simulink model "hopper_6dof_NED_v2_simplified"  (R2026a)
settings: Solver=FixedStepAuto  StopTime=30  FixedStep=1e-3  RelTol=1e-5
InitFcn:
  | % Feature toggles (1 = on, 0 = off). If no setup script defined them, default to
  | % full physics so this model always compiles and never silently drops physics.
  | % To turn a feature off for one run, prefer Simulink.SimulationInput.setVariable.
  | if ~exist('enable_slosh', 'var'), enable_slosh = 1; end
  | if ~exist('enable_wind', 'var'),  enable_wind  = 1; end
undefined symbols (not defined in the file): cg_init, dcg_dMfu_table, dcg_dMox_table, dI_dMfu_table, dI_dMox_table, ENGINE, engine_cg, engine_mass, fu_axial_damping_ratios, fu_lateral_damping_ratios, fu_mass_profile, fu_masses, fu_mdot_data, g, IN, K1flat, K2grid, MoI_init, mount_cg, OUT, ox_axial_damping_ratios, ox_lateral_damping_ratios, ox_mass_profile, ox_masses, ox_mdot_data, pressureLevels, r_leg_1, r_leg_2, r_leg_3, r_leg_4, tank_r, TANKS, Target_Trajectory, tgrid, thrust_data, unom, uwndTable, VEH, vwndTable
libraries: fl_lib x31, nesl_utility x25, matrix_library x18, SimscapeFluids_lib x10, simulink_extras x7, slpidlib x7, simulink x5, dspindex x3, sl_discontinuities x2, aerolibanim x1, commrandsrc3 x1, dspsrcs4 x1
(part 6 of 7)

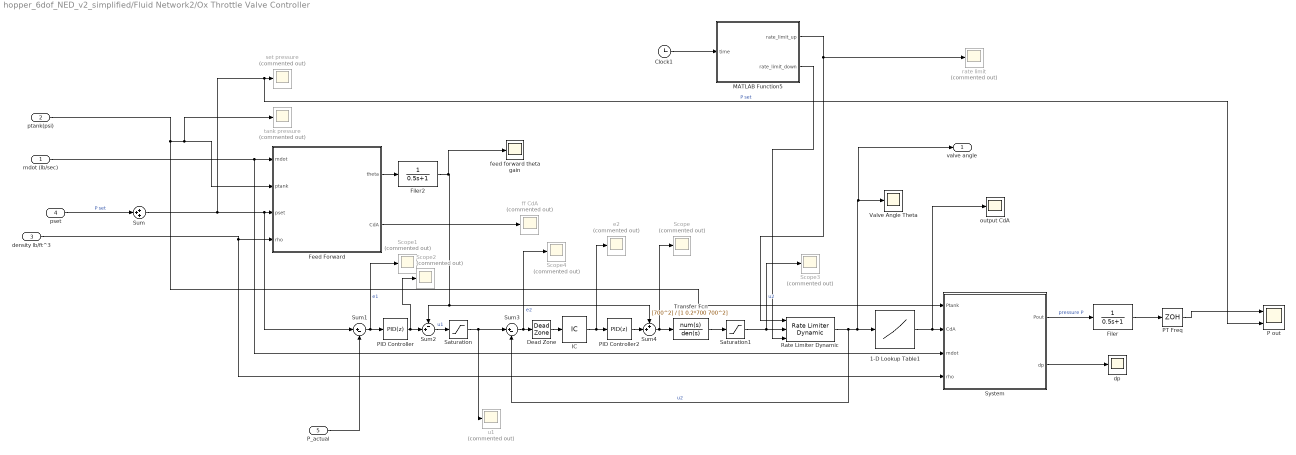
== system hopper_6dof_NED_v2_simplified/Fluid Network2/Ox Throttle Valve Controller ==
  mdot (lb/sec) : Inport
  ptank(psi) : Inport  Port=2
  density lb/ft^3 : Inport  Port=3
  pset : Inport  Port=4
  P_actual : Inport  Port=5
  1-D Lookup Table1 : Lookup_n-D  NumberOfTableDimensions=1  BreakpointsForDimension1=[27, 36, 45, 54, 63, 72, 81, 90]  Table="[0.01,  0.06, 0.21, 0.46, 0.83, 1.35, 2.04, 2.93] ./ 37.97"  ExtrapMethod=Clip  InternalRulePriority=Speed  RndMeth=Simplest
  Clock1 : Clock
  Dead Zone : DeadZone  LowerValue=-30  UpperValue=30
  Feed Forward : MATLAB Function  TreatAsAtomicUnit=on
  Filer : TransferFcn  Denominator=[0.5 1]
  Filer2 : TransferFcn  Denominator=[0.5 1]
  IC : InitialCondition  Value=0
  MATLAB Function5 : MATLAB Function  TreatAsAtomicUnit=on
  P out : Scope  NumInputPorts=2
      settings: ActiveDisplayYMinimum=-153.57845403205533  ActiveDisplayYMaximum=515.02423080214487  DataLoggingVariableName=ScopeData20
  PID Controller : slpidlib/PID Controller  Controller=PID  Form=Parallel  TimeDomain=Discrete-time  UseExternalTs=off  SampleTime=0.01  IntegratorMethod=Forward Euler  FilterMethod=Forward Euler  ControllerParametersSource=internal  P=6  I=0.5  UseKiTs=off  D=0  UseExternalDerivativeSource=off  N=100  UseFilter=on  TunerSelectOption=Transfer Function Based (PID Tuner App)  InitialConditionSource=internal  InitialConditionForIntegrator=0  InitialConditionForFilter=0  DifferentiatorICPrevScaledInput=0  ExternalReset=none  TrackingMode=off  Kt=1  LimitOutput=off  SatLimitsSource=internal  UpperSaturationLimit=inf  LowerSaturationLimit=-inf  LinearizeAsGain=on  AntiWindupMode=none  Kb=1  LimitIntegrator=off  UpperIntegratorSaturationLimit=inf  LowerIntegratorSaturationLimit=-inf  POutMin=[]  POutMax=[]  IOutMin=[]  IOutMax=[]  DOutMin=[]  DOutMax=[]  NOutMin=[]  NOutMax=[]  SumOutMin=[]  SumOutMax=[]  SaturationOutMin=[]  SaturationOutMax=[]  PParamMin=[]  PParamMax=[]  IParamMin=[]  IParamMax=[]  DParamMin=[]  DParamMax=[]  NParamMin=[]  NParamMax=[]  KbParamMin=[]  KbParamMax=[]  KtParamMin=[]  KtParamMax=[]  KbOutMin=[]  KbOutMax=[]  KtOutMin=[]  KtOutMax=[]  IntegratorOutMin=[]  IntegratorOutMax=[]  FilterOutMin=[]  FilterOutMax=[]  SumI1OutMin=[]  SumI1OutMax=[]  SumI2OutMin=[]  SumI2OutMax=[]  SumI3OutMin=[]  SumI3OutMax=[]  SumI4OutMin=[]  SumI4OutMax=[]  SumDOutMin=[]  SumDOutMax=[]  DifferentiatorOutMin=[]  DifferentiatorOutMax=[]  FilterDiffOutCoefMin=[]  FilterDiffOutCoefMax=[]  ReciprocalOutMin=[]  ReciprocalOutMax=[]  SumDenOutMin=[]  SumDenOutMax=[]  SumNumOutMin=[]  SumNumOutMax=[]  DivideOutMin=[]  DivideOutMax=[]  UdiffTsProdOutMin=[]  UdiffTsProdOutMax=[]  NTsProdOutMin=[]  NTsProdOutMax=[]  UintegralTsProdOutMin=[]  UintegralTsProdOutMax=[]  UngainTsProdOutMin=[]  UngainTsProdOutMax=[]  ClampingZeroOutDataTypeStr=Inherit: Inherit via back propagation  ClampingZeroOutMin=[]  ClampingZeroOutMax=[]  FilterDenConstantOutDataTypeStr=Inherit: Inherit via back propagation  FilterDenConstantOutMin=[]  FilterDenConstantOutMax=[]  PCopyOutDataTypeStr=Inherit: Inherit via back propagation  PCopyOutMin=[]  PCopyOutMax=[]  NCopyOutDataTypeStr=Inherit: Inherit via back propagation  NCopyOutMin=[]  NCopyOutMax=[]  IntegratorContinuousStateAttributes=''  IntegratorStateMustResolveToSignalObject=off  IntegratorRTWStateStorageClass=Auto  FilterContinuousStateAttributes=''  FilterStateMustResolveToSignalObject=off  FilterRTWStateStorageClass=Auto  ParallelPVariant=InternalParameters  IdealPVariant=Disabled  IVariant=InternalParameters  DVariant=InternalParameters  IntegratorVariant=Discrete  SatVariant=Disabled  AWVariant=Passthrough  PCopyVariant=Disabled  TRVariant=Disabled  FdbkBlocksVariant=Forward  IdealPFdbkVariant=Disabled  SatFdbkVariant=Disabled  DerivativeFilterVariant=ForwardEulerFilter  NVariant=InternalParameters  NCopyVariant=Disabled  FilterICVariant=InternalICsFilter  IntegratorICVariant=InternalICs  ExternalResetVariant=Disabled  TRSumVariant=Passthrough  SumFdbkVariant=Disabled  SumVariant=Sum_PID  TsampFilterVariant=InternalTs  TsampNgainVariant=Passthrough  TsampIntegralVariant=Disabled_SignalSpec  ExternalSaturationOutDataTypeStr=Inherit: Same as second input  DerivativeSourceVariant=ErrorSignal  PreIntVariant=InternalPreInt
  PID Controller2 : slpidlib/PID Controller  Controller=PID  Form=Parallel  TimeDomain=Discrete-time  UseExternalTs=off  SampleTime=0.001  IntegratorMethod=Forward Euler  FilterMethod=Forward Euler  ControllerParametersSource=internal  P=0.1  I=0.6  UseKiTs=off  D=0  UseExternalDerivativeSource=off  N=100  UseFilter=on  TunerSelectOption=Transfer Function Based (PID Tuner App)  InitialConditionSource=internal  InitialConditionForIntegrator=0  InitialConditionForFilter=0  DifferentiatorICPrevScaledInput=0  ExternalReset=none  TrackingMode=off  Kt=1  LimitOutput=off  SatLimitsSource=internal  UpperSaturationLimit=inf  LowerSaturationLimit=-inf  LinearizeAsGain=on  AntiWindupMode=none  Kb=1  LimitIntegrator=off  UpperIntegratorSaturationLimit=inf  LowerIntegratorSaturationLimit=-inf  POutMin=[]  POutMax=[]  IOutMin=[]  IOutMax=[]  DOutMin=[]  DOutMax=[]  NOutMin=[]  NOutMax=[]  SumOutMin=[]  SumOutMax=[]  SaturationOutMin=[]  SaturationOutMax=[]  PParamMin=[]  PParamMax=[]  IParamMin=[]  IParamMax=[]  DParamMin=[]  DParamMax=[]  NParamMin=[]  NParamMax=[]  KbParamMin=[]  KbParamMax=[]  KtParamMin=[]  KtParamMax=[]  KbOutMin=[]  KbOutMax=[]  KtOutMin=[]  KtOutMax=[]  IntegratorOutMin=[]  IntegratorOutMax=[]  FilterOutMin=[]  FilterOutMax=[]  SumI1OutMin=[]  SumI1OutMax=[]  SumI2OutMin=[]  SumI2OutMax=[]  SumI3OutMin=[]  SumI3OutMax=[]  SumI4OutMin=[]  SumI4OutMax=[]  SumDOutMin=[]  SumDOutMax=[]  DifferentiatorOutMin=[]  DifferentiatorOutMax=[]  FilterDiffOutCoefMin=[]  FilterDiffOutCoefMax=[]  ReciprocalOutMin=[]  ReciprocalOutMax=[]  SumDenOutMin=[]  SumDenOutMax=[]  SumNumOutMin=[]  SumNumOutMax=[]  DivideOutMin=[]  DivideOutMax=[]  UdiffTsProdOutMin=[]  UdiffTsProdOutMax=[]  NTsProdOutMin=[]  NTsProdOutMax=[]  UintegralTsProdOutMin=[]  UintegralTsProdOutMax=[]  UngainTsProdOutMin=[]  UngainTsProdOutMax=[]  ClampingZeroOutDataTypeStr=Inherit: Inherit via back propagation  ClampingZeroOutMin=[]  ClampingZeroOutMax=[]  FilterDenConstantOutDataTypeStr=Inherit: Inherit via back propagation  FilterDenConstantOutMin=[]  FilterDenConstantOutMax=[]  PCopyOutDataTypeStr=Inherit: Inherit via back propagation  PCopyOutMin=[]  PCopyOutMax=[]  NCopyOutDataTypeStr=Inherit: Inherit via back propagation  NCopyOutMin=[]  NCopyOutMax=[]  IntegratorContinuousStateAttributes=''  IntegratorStateMustResolveToSignalObject=off  IntegratorRTWStateStorageClass=Auto  FilterContinuousStateAttributes=''  FilterStateMustResolveToSignalObject=off  FilterRTWStateStorageClass=Auto  ParallelPVariant=InternalParameters  IdealPVariant=Disabled  IVariant=InternalParameters  DVariant=InternalParameters  IntegratorVariant=Discrete  SatVariant=Disabled  AWVariant=Passthrough  PCopyVariant=Disabled  TRVariant=Disabled  FdbkBlocksVariant=Forward  IdealPFdbkVariant=Disabled  SatFdbkVariant=Disabled  DerivativeFilterVariant=ForwardEulerFilter  NVariant=InternalParameters  NCopyVariant=Disabled  FilterICVariant=InternalICsFilter  IntegratorICVariant=InternalICs  ExternalResetVariant=Disabled  TRSumVariant=Passthrough  SumFdbkVariant=Disabled  SumVariant=Sum_PID  TsampFilterVariant=InternalTs  TsampNgainVariant=Passthrough  TsampIntegralVariant=Disabled_SignalSpec  ExternalSaturationOutDataTypeStr=Inherit: Same as second input  DerivativeSourceVariant=ErrorSignal  PreIntVariant=InternalPreInt
  PT Freq : ZeroOrderHold  SampleTime=1/200
  Rate Limiter Dynamic : sl_discontinuities/Rate Limiter Dynamic
  Saturation : Saturate  UpperLimit=90  LowerLimit=0
  Saturation1 : Saturate  UpperLimit=90  LowerLimit=0
  Scope{,1..4} (5 alike) : Scope  Commented=on
      Scope settings: ActiveDisplayYMinimum=-275.11641924282065  ActiveDisplayYMaximum=563.35245614782866  DataLoggingVariableName=ScopeData23
      Scope1 settings: ActiveDisplayYMinimum=-63.640747784829  ActiveDisplayYMaximum=395.9600830872032  DataLoggingVariableName=ScopeData24
      Scope2 settings: ActiveDisplayYMinimum=-1  ActiveDisplayYMaximum=1  DataLoggingVariableName=ScopeData25
      Scope3 settings: ActiveDisplayYMinimum=-1  ActiveDisplayYMaximum=1  DataLoggingVariableName=ScopeData26
      Scope4 settings: ActiveDisplayYMinimum=-1  ActiveDisplayYMaximum=1  DataLoggingVariableName=ScopeData27
  Sum : Sum  Inputs=+++
  Sum1 : Sum  Inputs=|+-
  Sum2 : Sum  Inputs=-+|
  Sum3 : Sum  Inputs=|+-
  Sum4 : Sum  Inputs=++|
  System : MATLAB Function  TreatAsAtomicUnit=on
  Transfer Fcn : TransferFcn  Numerator=[700^2]  Denominator=[1 0.2*700 700^2]
  Valve Angle Theta : Scope
      settings: ActiveDisplayYMinimum=-54.50975234839  ActiveDisplayYMaximum=77.0496336171224
  dp : Scope
      settings: ActiveDisplayYMinimum=-18119.240749435841  ActiveDisplayYMaximum=163753.70976632342  DataLoggingVariableName=ScopeData28
  e2 : Scope  Commented=on
      settings: ActiveDisplayYMinimum=-94.713391249832966  ActiveDisplayYMaximum=253.61308310962266  DataLoggingVariableName=ScopeData29
  feed forward theta gain : Scope
      settings: ActiveDisplayYMinimum=36.144112332478429  ActiveDisplayYMaximum=40.8018145520034  DataLoggingVariableName=ScopeData2
  ff CdA : Scope  Commented=on
      settings: ActiveDisplayYMinimum=0.00619  ActiveDisplayYMaximum=0.00757  DataLoggingVariableName=ScopeData30
  output CdA : Scope
      settings: ActiveDisplayYMinimum=-0.0014226243070618195  ActiveDisplayYMaximum=0.015437276914728357  DataLoggingVariableName=ScopeData3
  rate limit : Scope  Commented=on
      settings: ActiveDisplayYMinimum=-1  ActiveDisplayYMaximum=1  DataLoggingVariableName=ScopeData31
  set pressure : Scope  Commented=on
      settings: ActiveDisplayYMinimum=-1  ActiveDisplayYMaximum=1  DataLoggingVariableName=ScopeData32
  tank pressure : Scope  Commented=on
      settings: ActiveDisplayYMinimum=243.75  ActiveDisplayYMaximum=306.25  DataLoggingVariableName=ScopeData33
  u1 : Scope  Commented=on
      settings: ActiveDisplayYMinimum=-1  ActiveDisplayYMaximum=1  DataLoggingVariableName=ScopeData34
  valve angle : Outport
  wires:
  Sum3/1 -> Dead Zone/1, Scope4/1  "e2"
  density lb/ft^3/1 -> System/4(rho), Feed Forward/4(rho)
  Filer/1 -> PT Freq/1
  Sum/1 -> P out/2, set pressure/1, Sum1/1, Feed Forward/3(pset)  "P set"
  ptank(psi)/1 -> System/1(Ptank), Feed Forward/2(ptank), tank pressure/1
  PID Controller/1 -> Scope2/1, Sum2/2
  PT Freq/1 -> P out/1
  Transfer Fcn/1 -> Saturation1/1
  IC/1 -> PID Controller2/1, e2/1
  Feed Forward/1(theta) -> Filer2/1
  MATLAB Function5/2(rate_limit_down) -> Rate Limiter Dynamic/3
  Dead Zone/1 -> IC/1
  Rate Limiter Dynamic/1 -> valve angle/1, Valve Angle Theta/1, 1-D Lookup Table1/1, Sum3/2  "u2"
  pset/1 -> Sum/2  "P set"
  Sum4/1 -> Scope/1, Transfer Fcn/1
  Saturation1/1 -> Scope3/1, Rate Limiter Dynamic/2  "u2"
  mdot (lb/sec)/1 -> System/3(mdot), Feed Forward/1(mdot)
  MATLAB Function5/1(rate_limit_up) -> Rate Limiter Dynamic/1, rate limit/1
  Clock1/1 -> MATLAB Function5/1(time)
  1-D Lookup Table1/1 -> System/2(CdA), output CdA/1
  PID Controller2/1 -> Sum4/2
  Sum1/1 -> Scope1/1, PID Controller/1  "e1"
  Sum2/1 -> Saturation/1  "u1"
  Feed Forward/2(CdA) -> ff CdA/1
  System/2(dp) -> dp/1
  Saturation/1 -> u1/1, Sum3/1
  System/1(Pout) -> Filer/1  "pressure P"
  Filer2/1 -> Sum4/1, Sum2/1, feed forward theta gain/1
  P_actual/1 -> Sum1/2

== system hopper_6dof_NED_v2_simplified/Fluid Network2/Physical Combustion Chamber ==
  pc : Inport
  Local Restriction (TL) : fl_lib/Thermal Liquid/Elements/Local Restriction (TL)  Commented=through  restriction_type=foundation.enum.restriction_type.fixed  restriction_area=0.001 m^2  min_area=1e-10 m^2  max_area=0.005 m^2  area=0.01 m^2  Cd=0.64  Re_c=150  pressure_recovery=true
  Local Restriction (TL)1 : fl_lib/Thermal Liquid/Elements/Local Restriction (TL)  Commented=through  restriction_type=foundation.enum.restriction_type.fixed  restriction_area=0.001 m^2  min_area=1e-10 m^2  max_area=0.005 m^2  area=0.01 m^2  Cd=0.64  Re_c=150  pressure_recovery=true
  Pressure Source (TL) : fl_lib/Thermal Liquid/Sources/Pressure Source (TL)  source_type=foundation.enum.constant_controlled.controlled  pressure_differential=0 MPa  power_spec=foundation.enum.power_spec.isentropic  area=0.01 m^2
  Pressure Source (TL)1 : fl_lib/Thermal Liquid/Sources/Pressure Source (TL)  source_type=foundation.enum.constant_controlled.controlled  pressure_differential=0 MPa  power_spec=foundation.enum.power_spec.isentropic  area=0.01 m^2
  Reservoir (TL) : fl_lib/Thermal Liquid/Elements/Reservoir (TL)  pressure_input=false  pressure_spec=foundation.enum.pressure_spec.atmospheric  reservoir_pressure=0.101325 MPa  temperature_input=false  reservoir_temperature=293.15 K  area=0.01 m^2  input_error_spec=foundation.enum.input_range_error.warn
  Reservoir (TL)1 : fl_lib/Thermal Liquid/Elements/Reservoir (TL)  pressure_input=false  pressure_spec=foundation.enum.pressure_spec.atmospheric  reservoir_pressure=0.101325 MPa  temperature_input=false  reservoir_temperature=100 K  area=0.01 m^2  input_error_spec=foundation.enum.input_range_error.warn
  Simulink-PS Converter1 : nesl_utility/Simulink-PS Converter  PhysicalDomain=network_engine_domain  SubClassName=ps_input  LeftPortType=input  RightPortType=output  PseudoPeriodic=off  Frequencies=[]  NoiseDistribution=none  NoiseParameters=[]  Unit=1  AffineConversion=off  FilteringAndDerivatives=filter  SimscapeFilterOrder=1  InputFilterTimeConstant=0.001  UdotUserProvided=0
  Simulink-PS Converter4 : nesl_utility/Simulink-PS Converter  PhysicalDomain=network_engine_domain  SubClassName=ps_input  LeftPortType=input  RightPortType=output  PseudoPeriodic=off  Frequencies=[]  NoiseDistribution=none  NoiseParameters=[]  Unit=1  AffineConversion=off  FilteringAndDerivatives=filter  SimscapeFilterOrder=1  InputFilterTimeConstant=0.001  UdotUserProvided=0
  fuel line : PMIOPort  Side=Right
  ox line : PMIOPort  Port=2  Side=Right
  wires:
  pc/1 -> Simulink-PS Converter1/1, Simulink-PS Converter4/1
  connections:
  Simulink-PS Converter4/RConn1 -- Pressure Source (TL)/LConn2
  Simulink-PS Converter1/RConn1 -- Pressure Source (TL)1/LConn2
  Local Restriction (TL)/LConn1 -- Pressure Source (TL)/LConn1
  Reservoir (TL)/LConn1 -- Local Restriction (TL)/RConn1
  fuel line/RConn1 -- Pressure Source (TL)/RConn1
  Local Restriction (TL)1/LConn1 -- Pressure Source (TL)1/LConn1
  Reservoir (TL)1/LConn1 -- Local Restriction (TL)1/RConn1
  Pressure Source (TL)1/RConn1 -- ox line/RConn1

== system hopper_6dof_NED_v2_simplified/Fluid Network2/fuel mdot feedback//corrections ==
  actual mdot : Inport
  commanded mdot : Inport  Port=2
  MR correction : Inport  Port=3
  PID Controller1 : slpidlib/PID Controller  Controller=PID  Form=Parallel  TimeDomain=Continuous-time  UseExternalTs=off  SampleTime=-1  IntegratorMethod=Forward Euler  FilterMethod=Forward Euler  ControllerParametersSource=internal  P=1  I=1  UseKiTs=off  D=0  UseExternalDerivativeSource=off  N=20  UseFilter=on  TunerSelectOption=Transfer Function Based (PID Tuner App)  InitialConditionSource=internal  InitialConditionForIntegrator=0  InitialConditionForFilter=0  DifferentiatorICPrevScaledInput=0  ExternalReset=none  TrackingMode=off  Kt=1  LimitOutput=off  SatLimitsSource=internal  UpperSaturationLimit=inf  LowerSaturationLimit=-inf  LinearizeAsGain=on  AntiWindupMode=none  Kb=1  LimitIntegrator=off  UpperIntegratorSaturationLimit=inf  LowerIntegratorSaturationLimit=-inf  POutMin=[]  POutMax=[]  IOutMin=[]  IOutMax=[]  DOutMin=[]  DOutMax=[]  NOutMin=[]  NOutMax=[]  SumOutMin=[]  SumOutMax=[]  SaturationOutMin=[]  SaturationOutMax=[]  PParamMin=[]  PParamMax=[]  IParamMin=[]  IParamMax=[]  DParamMin=[]  DParamMax=[]  NParamMin=[]  NParamMax=[]  KbParamMin=[]  KbParamMax=[]  KtParamMin=[]  KtParamMax=[]  KbOutMin=[]  KbOutMax=[]  KtOutMin=[]  KtOutMax=[]  IntegratorOutMin=[]  IntegratorOutMax=[]  FilterOutMin=[]  FilterOutMax=[]  SumI1OutMin=[]  SumI1OutMax=[]  SumI2OutMin=[]  SumI2OutMax=[]  SumI3OutMin=[]  SumI3OutMax=[]  SumI4OutMin=[]  SumI4OutMax=[]  SumDOutMin=[]  SumDOutMax=[]  DifferentiatorOutMin=[]  DifferentiatorOutMax=[]  FilterDiffOutCoefMin=[]  FilterDiffOutCoefMax=[]  ReciprocalOutMin=[]  ReciprocalOutMax=[]  SumDenOutMin=[]  SumDenOutMax=[]  SumNumOutMin=[]  SumNumOutMax=[]  DivideOutMin=[]  DivideOutMax=[]  UdiffTsProdOutMin=[]  UdiffTsProdOutMax=[]  NTsProdOutMin=[]  NTsProdOutMax=[]  UintegralTsProdOutMin=[]  UintegralTsProdOutMax=[]  UngainTsProdOutMin=[]  UngainTsProdOutMax=[]  ClampingZeroOutDataTypeStr=Inherit: Inherit via back propagation  ClampingZeroOutMin=[]  ClampingZeroOutMax=[]  FilterDenConstantOutDataTypeStr=Inherit: Inherit via back propagation  FilterDenConstantOutMin=[]  FilterDenConstantOutMax=[]  PCopyOutDataTypeStr=Inherit: Inherit via back propagation  PCopyOutMin=[]  PCopyOutMax=[]  NCopyOutDataTypeStr=Inherit: Inherit via back propagation  NCopyOutMin=[]  NCopyOutMax=[]  IntegratorContinuousStateAttributes=''  IntegratorStateMustResolveToSignalObject=off  IntegratorRTWStateStorageClass=Auto  FilterContinuousStateAttributes=''  FilterStateMustResolveToSignalObject=off  FilterRTWStateStorageClass=Auto  ParallelPVariant=InternalParameters  IdealPVariant=Disabled  IVariant=InternalParameters  DVariant=InternalParameters  IntegratorVariant=Continuous  SatVariant=Disabled  AWVariant=Passthrough  PCopyVariant=Disabled  TRVariant=Disabled  FdbkBlocksVariant=Forward  IdealPFdbkVariant=Disabled  SatFdbkVariant=Disabled  DerivativeFilterVariant=ContFilter  NVariant=InternalParameters  NCopyVariant=Disabled  FilterICVariant=InternalICsFilter  IntegratorICVariant=InternalICs  ExternalResetVariant=Disabled  TRSumVariant=Passthrough  SumFdbkVariant=Disabled  SumVariant=Sum_PID  TsampFilterVariant=InternalTs  TsampNgainVariant=Passthrough  TsampIntegralVariant=Disabled_SignalSpec  ExternalSaturationOutDataTypeStr=Inherit: Same as second input  DerivativeSourceVariant=ErrorSignal  PreIntVariant=InternalPreInt
  Sum2 : Sum  Inputs=|+-
  Sum3 : Sum  Inputs=|+-
  Sum4 : Sum  Inputs=|++
  kg/s to lb/s1 : Gain  Gain=2.20462
  fuel mdot : Outport
  wires:
  MR correction/1 -> Sum2/2
  Sum2/1 -> Sum4/2, Sum3/1
  PID Controller1/1 -> Sum4/1
  Sum3/1 -> PID Controller1/1
  Sum4/1 -> kg/s to lb/s1/1
  commanded mdot/1 -> Sum2/1
  actual mdot/1 -> Sum3/2
  kg/s to lb/s1/1 -> fuel mdot/1

== system hopper_6dof_NED_v2_simplified/Fluid Network2/ox mdot feedback//corrections ==
  commanded mdot : Inport
  actual mdot : Inport  Port=2
  PID Controller2 : slpidlib/PID Controller  Controller=PID  Form=Parallel  TimeDomain=Continuous-time  UseExternalTs=off  SampleTime=-1  IntegratorMethod=Forward Euler  FilterMethod=Forward Euler  ControllerParametersSource=internal  P=1  I=1  UseKiTs=off  D=0  UseExternalDerivativeSource=off  N=20  UseFilter=on  TunerSelectOption=Transfer Function Based (PID Tuner App)  InitialConditionSource=internal  InitialConditionForIntegrator=0  InitialConditionForFilter=0  DifferentiatorICPrevScaledInput=0  ExternalReset=none  TrackingMode=off  Kt=1  LimitOutput=off  SatLimitsSource=internal  UpperSaturationLimit=inf  LowerSaturationLimit=-inf  LinearizeAsGain=on  AntiWindupMode=none  Kb=1  LimitIntegrator=off  UpperIntegratorSaturationLimit=inf  LowerIntegratorSaturationLimit=-inf  POutMin=[]  POutMax=[]  IOutMin=[]  IOutMax=[]  DOutMin=[]  DOutMax=[]  NOutMin=[]  NOutMax=[]  SumOutMin=[]  SumOutMax=[]  SaturationOutMin=[]  SaturationOutMax=[]  PParamMin=[]  PParamMax=[]  IParamMin=[]  IParamMax=[]  DParamMin=[]  DParamMax=[]  NParamMin=[]  NParamMax=[]  KbParamMin=[]  KbParamMax=[]  KtParamMin=[]  KtParamMax=[]  KbOutMin=[]  KbOutMax=[]  KtOutMin=[]  KtOutMax=[]  IntegratorOutMin=[]  IntegratorOutMax=[]  FilterOutMin=[]  FilterOutMax=[]  SumI1OutMin=[]  SumI1OutMax=[]  SumI2OutMin=[]  SumI2OutMax=[]  SumI3OutMin=[]  SumI3OutMax=[]  SumI4OutMin=[]  SumI4OutMax=[]  SumDOutMin=[]  SumDOutMax=[]  DifferentiatorOutMin=[]  DifferentiatorOutMax=[]  FilterDiffOutCoefMin=[]  FilterDiffOutCoefMax=[]  ReciprocalOutMin=[]  ReciprocalOutMax=[]  SumDenOutMin=[]  SumDenOutMax=[]  SumNumOutMin=[]  SumNumOutMax=[]  DivideOutMin=[]  DivideOutMax=[]  UdiffTsProdOutMin=[]  UdiffTsProdOutMax=[]  NTsProdOutMin=[]  NTsProdOutMax=[]  UintegralTsProdOutMin=[]  UintegralTsProdOutMax=[]  UngainTsProdOutMin=[]  UngainTsProdOutMax=[]  ClampingZeroOutDataTypeStr=Inherit: Inherit via back propagation  ClampingZeroOutMin=[]  ClampingZeroOutMax=[]  FilterDenConstantOutDataTypeStr=Inherit: Inherit via back propagation  FilterDenConstantOutMin=[]  FilterDenConstantOutMax=[]  PCopyOutDataTypeStr=Inherit: Inherit via back propagation  PCopyOutMin=[]  PCopyOutMax=[]  NCopyOutDataTypeStr=Inherit: Inherit via back propagation  NCopyOutMin=[]  NCopyOutMax=[]  IntegratorContinuousStateAttributes=''  IntegratorStateMustResolveToSignalObject=off  IntegratorRTWStateStorageClass=Auto  FilterContinuousStateAttributes=''  FilterStateMustResolveToSignalObject=off  FilterRTWStateStorageClass=Auto  ParallelPVariant=InternalParameters  IdealPVariant=Disabled  IVariant=InternalParameters  DVariant=InternalParameters  IntegratorVariant=Continuous  SatVariant=Disabled  AWVariant=Passthrough  PCopyVariant=Disabled  TRVariant=Disabled  FdbkBlocksVariant=Forward  IdealPFdbkVariant=Disabled  SatFdbkVariant=Disabled  DerivativeFilterVariant=ContFilter  NVariant=InternalParameters  NCopyVariant=Disabled  FilterICVariant=InternalICsFilter  IntegratorICVariant=InternalICs  ExternalResetVariant=Disabled  TRSumVariant=Passthrough  SumFdbkVariant=Disabled  SumVariant=Sum_PID  TsampFilterVariant=InternalTs  TsampNgainVariant=Passthrough  TsampIntegralVariant=Disabled_SignalSpec  ExternalSaturationOutDataTypeStr=Inherit: Same as second input  DerivativeSourceVariant=ErrorSignal  PreIntVariant=InternalPreInt
  Sum1 : Sum  Inputs=|+-
  Sum5 : Sum  Inputs=|++
  kg/s to lb/s : Gain  Gain=2.20462
  ox mdot : Outport
  wires:
  Sum1/1 -> PID Controller2/1
  commanded mdot/1 -> Sum5/2, Sum1/1
  PID Controller2/1 -> Sum5/1
  Sum5/1 -> kg/s to lb/s/1
  kg/s to lb/s/1 -> ox mdot/1
  actual mdot/1 -> Sum1/2

== system hopper_6dof_NED_v2_simplified/Ground /Leg 1 Force ==
  Leg Position : Inport
  Leg Velocity : Inport  Port=2
  Demux : Demux  Outputs=3
  Demux1 : Demux  Outputs=3
  If : If  NumInputs=2  IfExpression=u1 > -0.001
  If Action Subsystem : Subsystem  TreatAsAtomicUnit=on
  If Action Subsystem1 : Subsystem  TreatAsAtomicUnit=on
  Merge : Merge
  Leg 1 Force : Outport
  wires:
  Leg Position/1 -> If Action Subsystem/1(Leg Position), Demux/1
  If/2 -> If Action Subsystem1/Action
  If Action Subsystem/1(Leg Force) -> Merge/1
  If Action Subsystem1/1(Out1) -> Merge/2
  Merge/1 -> Leg 1 Force/1
  Leg Velocity/1 -> Demux1/1, If Action Subsystem/2(Leg Velocity)
  If/1 -> If Action Subsystem/Action
  Demux/3 -> If/1
  Demux1/3 -> If/2

== system hopper_6dof_NED_v2_simplified/Ground /Leg 1 Force1 ==
  Leg Position : Inport
  Leg Velocity : Inport  Port=2
  Demux : Demux  Outputs=3
  Demux1 : Demux  Outputs=3
  If : If  NumInputs=2  IfExpression=u1 > -0.001
  If Action Subsystem : Subsystem  TreatAsAtomicUnit=on
  If Action Subsystem1 : Subsystem  TreatAsAtomicUnit=on
  Merge : Merge
  Leg 1 Force : Outport
  wires:
  Leg Position/1 -> If Action Subsystem/1(Leg Position), Demux/1
  If/2 -> If Action Subsystem1/Action
  If Action Subsystem/1(Leg Force) -> Merge/1
  If Action Subsystem1/1(Out1) -> Merge/2
  Merge/1 -> Leg 1 Force/1
  Leg Velocity/1 -> Demux1/1, If Action Subsystem/2(Leg Velocity)
  If/1 -> If Action Subsystem/Action
  Demux/3 -> If/1
  Demux1/3 -> If/2

== system hopper_6dof_NED_v2_simplified/Ground /Leg 1 Force2 ==
  Leg Position : Inport
  Leg Velocity : Inport  Port=2
  Demux : Demux  Outputs=3
  Demux1 : Demux  Outputs=3
  If : If  NumInputs=2  IfExpression=u1 > -0.001
  If Action Subsystem : Subsystem  TreatAsAtomicUnit=on
  If Action Subsystem1 : Subsystem  TreatAsAtomicUnit=on
  Merge : Merge
  Leg 1 Force : Outport
  wires:
  Leg Position/1 -> If Action Subsystem/1(Leg Position), Demux/1
  If/2 -> If Action Subsystem1/Action
  If Action Subsystem/1(Leg Force) -> Merge/1
  If Action Subsystem1/1(Out1) -> Merge/2
  Merge/1 -> Leg 1 Force/1
  Leg Velocity/1 -> Demux1/1, If Action Subsystem/2(Leg Velocity)
  If/1 -> If Action Subsystem/Action
  Demux/3 -> If/1
  Demux1/3 -> If/2

== system hopper_6dof_NED_v2_simplified/Ground /Leg 1 Force3 ==
  Leg Position : Inport
  Leg Velocity : Inport  Port=2
  Demux : Demux  Outputs=3
  Demux1 : Demux  Outputs=3
  If : If  NumInputs=2  IfExpression=u1 > -0.001
  If Action Subsystem : Subsystem  TreatAsAtomicUnit=on
  If Action Subsystem1 : Subsystem  TreatAsAtomicUnit=on
  Merge : Merge
  Leg 1 Force : Outport
  wires:
  Leg Position/1 -> If Action Subsystem/1(Leg Position), Demux/1
  If/2 -> If Action Subsystem1/Action
  If Action Subsystem/1(Leg Force) -> Merge/1
  If Action Subsystem1/1(Out1) -> Merge/2
  Merge/1 -> Leg 1 Force/1
  Leg Velocity/1 -> Demux1/1, If Action Subsystem/2(Leg Velocity)
  If/1 -> If Action Subsystem/Action
  Demux/3 -> If/1
  Demux1/3 -> If/2

== system hopper_6dof_NED_v2_simplified/Gusts/Disabled ==
  Zero1 : Constant  Value=0
  Out1 : Outport
  wires:
  Zero1/1 -> Out1/1

== system hopper_6dof_NED_v2_simplified/Gusts/Enabled ==
  Bernoulli Binary Generator : commrandsrc3/Bernoulli Binary Generator  ProbabilityOfZero=0.95  SeedSource=Parameter  Seed=0  SampleTime=0.1  SamplesPerFrame=1  OutputDataType=double  SimulateUsing=Interpreted execution
  Product1 : Product
  Random Source : dspsrcs4/Random Source  SrcType=Gaussian  MinVal=0  MaxVal=1  MeanVal=0  VarVal=20  RepMode=Specify seed  rawSeed=1  IsInherit=off  SampTime=1  SampFrame=1  OutComplex=Real  DataType=double  SimulateUsing=Interpreted execution
  Out1 : Outport
  wires:
  Product1/1 -> Out1/1
  Bernoulli Binary Generator/1 -> Product1/1
  Random Source/1 -> Product1/2

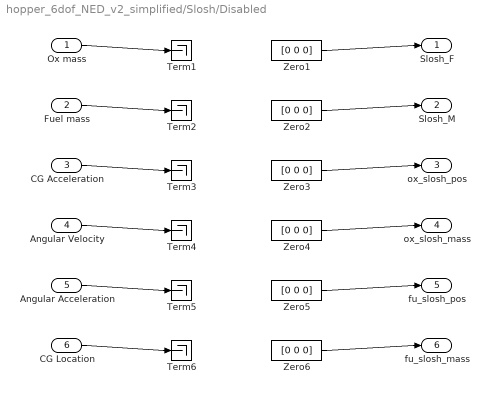
== system hopper_6dof_NED_v2_simplified/Slosh/Disabled ==
  Ox mass : Inport
  Fuel mass : Inport  Port=2
  CG Acceleration : Inport  Port=3
  Angular Velocity : Inport  Port=4
  Angular Acceleration : Inport  Port=5
  CG Location : Inport  Port=6
  Term{1..6} (6 alike) : Terminator
  Zero{1..6} (6 alike) : Constant  Value=[0 0 0]
  Slosh_F : Outport
  Slosh_M : Outport  Port=2
  ox_slosh_pos : Outport  Port=3
  ox_slosh_mass : Outport  Port=4
  fu_slosh_pos : Outport  Port=5
  fu_slosh_mass : Outport  Port=6
  wires:
  Ox mass/1 -> Term1/1
  Fuel mass/1 -> Term2/1
  CG Acceleration/1 -> Term3/1
  Angular Velocity/1 -> Term4/1
  Angular Acceleration/1 -> Term5/1
  CG Location/1 -> Term6/1
  Zero1/1 -> Slosh_F/1
  Zero2/1 -> Slosh_M/1
  Zero3/1 -> ox_slosh_pos/1
  Zero4/1 -> ox_slosh_mass/1
  Zero5/1 -> fu_slosh_pos/1
  Zero6/1 -> fu_slosh_mass/1

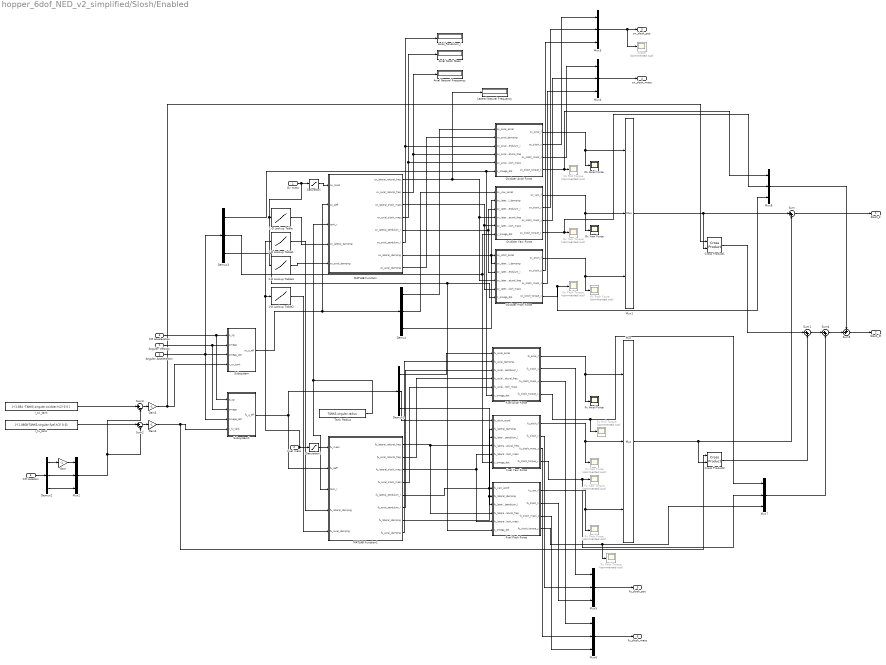
== system hopper_6dof_NED_v2_simplified/Slosh/Enabled ==
  Ox mass : Inport
  Fuel mass : Inport  Port=2
  CG Acceleration : Inport  Port=3
  Angular Velocity : Inport  Port=4
  Angular Acceleration : Inport  Port=5
  CG Location : Inport  Port=6
  1-D Lookup Table : Lookup_n-D  NumberOfTableDimensions=1  BreakpointsForDimension1=ox_mass_profile  Table=ox_lateral_damping_ratios  InternalRulePriority=Speed  RndMeth=Simplest
  1-D Lookup Table1 : Lookup_n-D  NumberOfTableDimensions=1  BreakpointsForDimension1=fu_mass_profile  Table=fu_lateral_damping_ratios  InternalRulePriority=Speed  RndMeth=Simplest
  1-D Lookup Table2 : Lookup_n-D  NumberOfTableDimensions=1  BreakpointsForDimension1=fu_mass_profile  Table=fu_axial_damping_ratios  InternalRulePriority=Speed  RndMeth=Simplest
  1-D Lookup Table4 : Lookup_n-D  NumberOfTableDimensions=1  BreakpointsForDimension1=ox_mass_profile  Table=ox_axial_damping_ratios  InternalRulePriority=Speed  RndMeth=Simplest
  Axial Natural Frequency : Display
  Axial Slosh Mass : Display
  Axial_Pendulum_l : Display
  Cross Product1 : matrix_library/Cross Product
  Cross Product2 : matrix_library/Cross Product
  Demux{,1..3} (4 alike) : Demux  Outputs=3
  Fu Axial Force : Scope
      settings: ActiveDisplayYMinimum=-4.5487995330933861  ActiveDisplayYMaximum=10.430303988696288  DataLoggingVariableName=ScopeData38
  Fu Pitch Force : Scope  Commented=on
      settings: ActiveDisplayYMinimum=-2.9742058993087932  ActiveDisplayYMaximum=15.331760127930639  DataLoggingVariableName=ScopeData40
  Fu Pitch Torque : Scope  Commented=on
      settings: ActiveDisplayYMinimum=-0.19116574787256713  ActiveDisplayYMaximum=0.19970427620804132  DataLoggingVariableName=ScopeData87
  Fu Roll Torque : Scope  Commented=on
      settings: ActiveDisplayYMinimum=-9.5580450498277436  ActiveDisplayYMaximum=8.6061310713641461  DataLoggingVariableName=ScopeData86
  Fu Yaw Force : Scope  Commented=on
      settings: ActiveDisplayYMinimum=-1.96682346554972  ActiveDisplayYMaximum=2.7427386100438831  DataLoggingVariableName=ScopeData39
  Fu Yaw Torque : Scope  Commented=on
      settings: ActiveDisplayYMinimum=-3.6886267521568623  ActiveDisplayYMaximum=3.9647425854021145  DataLoggingVariableName=ScopeData82
  Fuel Axial Force : Subsystem
  Fuel Pitch Force : Subsystem
  Fuel Yaw Force : Subsystem
  Gain : Gain  Gain=-1
  Gain3 : Gain  Gain=-1
  Gain4 : Gain  Gain=-1
  Lateral Natural Frequency : Display
  MATLAB Function : MATLAB Function  TreatAsAtomicUnit=on
  MATLAB Function1 : MATLAB Function  TreatAsAtomicUnit=on
  Mux{,1..8} (9 alike) : Mux  Inputs=3
  Ox Axial Force : Scope
      settings: ActiveDisplayYMinimum=14.43010515330246  ActiveDisplayYMaximum=16.756383333748122  DataLoggingVariableName=ScopeData34
  Ox Pitch Force : Scope  Commented=on
      settings: ActiveDisplayYMinimum=-4.4950785008236629  ActiveDisplayYMaximum=22.001881619828325  DataLoggingVariableName=ScopeData36
  Ox Pitch Torque : Scope  Commented=on
      settings: ActiveDisplayYMinimum=-0.69593653498138675  ActiveDisplayYMaximum=0.79680864639954685  DataLoggingVariableName=ScopeData85
  Ox Roll Torque : Scope  Commented=on
      settings: ActiveDisplayYMinimum=-0.15656949128956149  ActiveDisplayYMaximum=0.79158034254760723  DataLoggingVariableName=ScopeData80
  Ox Yaw Force : Scope
      settings: ActiveDisplayYMinimum=-5.8284827308381395  ActiveDisplayYMaximum=24.723450598791928  DataLoggingVariableName=ScopeData37
  Ox Yaw Torque : Scope  Commented=on
      settings: ActiveDisplayYMinimum=-0.3482323750211066  ActiveDisplayYMaximum=0.31743853430357161  DataLoggingVariableName=ScopeData81
  Oxidizer Axial Force : Subsystem
  Oxidizer Pitch Force : Subsystem
  Oxidizer Yaw Force : Subsystem
  Saturation : Saturate  UpperLimit=inf  LowerLimit=0.01
  Saturation1 : Saturate  UpperLimit=inf  LowerLimit=0.01
  Scope : Scope  Commented=on
      settings: ActiveDisplayYMinimum=-0.0849364779794028  ActiveDisplayYMaximum=0.368207880424993  DataLoggingVariableName=ScopeData35
  Subsystem : Subsystem
  Subsystem1 : Subsystem
  Sum : Sum  Inputs=|++
  Sum1 : Sum  Inputs=|++
  Sum2 : Sum  Inputs=|+-
  Sum3 : Sum  Inputs=|+-
  Sum4 : Sum  Inputs=|++
  Sum5 : Sum  Inputs=++|
  Tank Radius : Constant  Value=TANKS.singular.radius  SampleTime=-1
  r_fu_tank : Constant  Value=[-(1.0668-TANKS.singular.fuel.h/2) 0 0]
  r_ox_tank : Constant  Value=[-(1.854 -TANKS.singular.oxidizer.h/2) 0 0 ]
  Slosh_F : Outport
  Slosh_M : Outport  Port=2
  ox_slosh_pos : Outport  Port=3
  ox_slosh_mass : Outport  Port=4
  fu_slosh_pos : Outport  Port=5
  fu_slosh_mass : Outport  Port=6
  wires:
  1-D Lookup Table2/1 -> MATLAB Function1/5("fu_axial_damping ")
  1-D Lookup Table4/1 -> MATLAB Function/5("ox_axial_damping ")
  1-D Lookup Table1/1 -> MATLAB Function1/4("fu_lateral_damping ")
  1-D Lookup Table/1 -> MATLAB Function/4("ox_lateral_damping ")
  Saturation1/1 -> MATLAB Function1/1(fu_mass)
  Saturation/1 -> MATLAB Function/1(ox_mass)
  Mux7/1 -> Sum4/2
  Mux8/1 -> Sum5/1
  Oxidizer Yaw Force/4(ox_slosh_torque_y) -> Ox Yaw Torque/1, Mux8/2
  Sum4/1 -> Sum5/2
  Sum5/1 -> Slosh_M/1
  Sum1/1 -> Sum4/1
  Oxidizer Pitch Force/4(ox_slosh_torque_z) -> Mux8/3, Ox Pitch Torque/1
  Oxidizer Axial Force/4(ox_slosh_torque_x) -> Ox Roll Torque/1, Mux8/1
  Fuel Pitch Force/4(fu_slosh_torque_z) -> Fu Pitch Torque/1, Mux7/3
  Fuel Yaw Force/4(fu_slosh_torque_y) -> Fu Yaw Torque/1, Mux7/2
  Fuel Axial Force/4(fu_slosh_torque_x) -> Fu Roll Torque/1, Mux7/1
  Demux3/3 -> Oxidizer Pitch Force/6(z_omega_dot), Fuel Pitch Force/6(z_omega_dot)
  Demux3/2 -> Oxidizer Yaw Force/6(y_omega_dot), Fuel Yaw Force/6(y_omega_dot)
  Demux3/1 -> Fuel Axial Force/6(x_omega_dot), Oxidizer Axial Force/6(x_omega_dot)
  Fuel Axial Force/2(fu_slosh_x) -> Mux5/1
  Oxidizer Axial Force/2(ox_slosh_x) -> Mux3/1
  Fuel Pitch Force/3(fu_slosh_mass_z) -> Mux6/3
  Fuel Yaw Force/3(fu_slosh_mass_y) -> Mux6/2
  Fuel Axial Force/3(fu_slosh_mass_x) -> Mux6/1
  Fuel Pitch Force/2(fu_slosh_z) -> Mux5/3
  Fuel Yaw Force/2(fu_slosh_y) -> Mux5/2
  Mux6/1 -> fu_slosh_mass/1
  Mux5/1 -> fu_slosh_pos/1
  Mux4/1 -> ox_slosh_mass/1
  Oxidizer Pitch Force/3(ox_slosh_mass_z) -> Mux4/3
  Oxidizer Pitch Force/2(ox_slosh_z) -> Mux3/3
  Oxidizer Yaw Force/3(ox_slosh_mass_y) -> Mux4/2
  Oxidizer Axial Force/3(ox_slosh_mass_x) -> Mux4/1
  Mux3/1 -> ox_slosh_pos/1, Scope/1
  Oxidizer Yaw Force/2(ox_slosh_y) -> Mux3/2
  Gain/1 -> Mux2/1
  Demux2/1 -> Gain/1
  Demux2/2 -> Mux2/2
  CG Location/1 -> Demux2/1
  Demux2/3 -> Mux2/3
  Gain4/1 -> Subsystem1/4(r_fu_tank), Cross Product2/1
  Gain3/1 -> Subsystem/4(r_ox_tank), Cross Product1/1
  Oxidizer Pitch Force/1(ox_pitch_f) -> Ox Pitch Force/1, Mux1/3
  Fuel Pitch Force/1(fu_yaw_f) -> Fu Pitch Force/1, Mux/3
  Sum2/1 -> Gain4/1
  Sum3/1 -> Gain3/1
  Mux2/1 -> Sum3/2, Sum2/2
  r_fu_tank/1 -> Sum2/1
  r_ox_tank/1 -> Sum3/1
  Tank Radius/1 -> MATLAB Function/3(tank_r), MATLAB Function1/3(tank_r)
  Cross Product2/1 -> Sum1/2
  Cross Product1/1 -> Sum1/1
  Sum/1 -> Slosh_F/1
  Mux/1 -> Cross Product2/2, Sum/2
  Mux1/1 -> Sum/1, Cross Product1/2
  Oxidizer Yaw Force/1(ox_yaw_f) -> Mux1/2, Ox Yaw Force/1
  Oxidizer Axial Force/1(ox_axial_f) -> Mux1/1, Ox Axial Force/1
  Fuel Yaw Force/1(fu_pitch_f) -> Mux/2, Fu Yaw Force/1
  Fuel Axial Force/1(fu_axial_f) -> Mux/1, Fu Axial Force/1
  MATLAB Function1/8(fu_axial_damping) -> Fuel Axial Force/2(fu_axial_damping)
  MATLAB Function1/7(fu_lateral_damping) -> Fuel Pitch Force/2(fu_lateral_damping), Fuel Yaw Force/2(fu_lateral_damping)
  MATLAB Function1/6(fu_axial_pendulum_l) -> Fuel Axial Force/3(fu_axial_pendulum_l)
  MATLAB Function1/5(fu_lateral_pendulum_l) -> Fuel Pitch Force/3(fu_lateral_pendulum_l), Fuel Yaw Force/3(fu_lateral_pendulum_l)
  MATLAB Function1/4(fu_axial_slosh_mass) -> Fuel Axial Force/5(fu_axial_slosh_mass)
  MATLAB Function1/3(fu_lateral_slosh_mass) -> Fuel Pitch Force/5(fu_lateral_slosh_mass), Fuel Yaw Force/5(fu_lateral_slosh_mass)
  MATLAB Function1/2(fu_axial_natural_freq) -> Fuel Axial Force/4(fu_axial_natural_freq)
  MATLAB Function1/1(fu_lateral_natural_freq) -> Fuel Yaw Force/4(fu_lateral_natural_freq), Fuel Pitch Force/4(fu_lateral_natural_freq)
  MATLAB Function/8(ox_axial_damping) -> Oxidizer Axial Force/2(ox_axial_damping)
  MATLAB Function/7(ox_lateral_damping) -> Oxidizer Pitch Force/2(ox_lateral_damping), Oxidizer Yaw Force/2(ox_lateral_damping)
  MATLAB Function/6(ox_axial_pendulum_l) -> Oxidizer Axial Force/3(ox_axial_pendulum_l), Axial_Pendulum_l/1
  MATLAB Function/5(ox_lateral_pendulum_l) -> Oxidizer Pitch Force/3(ox_lateral_pendulum_l), Oxidizer Yaw Force/3(ox_lateral_pendulum_l)
  MATLAB Function/4(ox_axial_slosh_mass) -> Oxidizer Axial Force/5(ox_axial_slosh_mass), Axial Slosh Mass/1
  MATLAB Function/3(ox_lateral_slosh_mass) -> Oxidizer Yaw Force/5(ox_lateral_slosh_mass), Oxidizer Pitch Force/5(ox_lateral_slosh_mass)
  MATLAB Function/2(ox_axial_natural_freq) -> Oxidizer Axial Force/4(ox_axial_natural_freq), Axial Natural Frequency/1
  MATLAB Function/1(ox_lateral_natural_freq) -> Oxidizer Yaw Force/4(ox_lateral_natural_freq), Oxidizer Pitch Force/4(ox_lateral_natural_freq), Lateral Natural Frequency/1
  Demux1/3 -> Fuel Pitch Force/1(fu_yaw_accel)
  Demux1/2 -> Fuel Yaw Force/1(fu_pitch_accel)
  Demux1/1 -> Fuel Axial Force/1(fu_axial_accel)
  Demux/3 -> Oxidizer Pitch Force/1(ox_pitch_accel)
  Demux/2 -> Oxidizer Yaw Force/1(ox_yaw_accel)
  Demux/1 -> Oxidizer Axial Force/1(ox_axial_accel)
  Subsystem1/1(fu_a_eff) -> MATLAB Function1/2(fu_aeff), Demux1/1
  Subsystem/1(ox_a_eff) -> MATLAB Function/2(ox_aeff), Demux/1
  Fuel mass/1 -> Saturation1/1, 1-D Lookup Table1/1, 1-D Lookup Table2/1
  Angular Acceleration/1 -> Demux3/1, Subsystem1/3(omega_dot), Subsystem/3(omega_dot)
  Angular Velocity/1 -> Subsystem1/2(omega), Subsystem/2(omega)
  CG Acceleration/1 -> Subsystem1/1(a_cg), Subsystem/1(a_cg)
  Ox mass/1 -> Saturation/1, 1-D Lookup Table/1, 1-D Lookup Table4/1

== system hopper_6dof_NED_v2_simplified/Subsystem2/If Action Subsystem ==
  Thrust : Inport
  Action Port : ActionPort  ActionPortLabel=if(u1 > 0 & u2 > 0)
  Out1 : Outport
  wires:
  Thrust/1 -> Out1/1

== system hopper_6dof_NED_v2_simplified/Subsystem2/If Action Subsystem1 ==
  Thrust : Inport
  Action Port : ActionPort  ActionPortLabel=else
  Gain : Gain  Gain=0
  Out1 : Outport
  wires:
  Thrust/1 -> Gain/1
  Gain/1 -> Out1/1

== system hopper_6dof_NED_v2_simplified/Subsystem3/If Action Subsystem ==
  In1 : Inport
  Action Port : ActionPort  ActionPortLabel=|
      | if(u1 > -1e-3 & u2 > 0
      | )
  Delay : Delay  Commented=through
  Stop Simulation : Stop
  wires:
  In1/1 -> Delay/1
  Delay/1 -> Stop Simulation/1

== system hopper_6dof_NED_v2_simplified/Subsystem4/If Action Subsystem ==
  Thrust : Inport
  Action Port : ActionPort  ActionPortLabel=else
  Out1 : Outport
  wires:
  Thrust/1 -> Out1/1

== system hopper_6dof_NED_v2_simplified/Subsystem4/If Action Subsystem1 ==
  Thrust : Inport
  Action Port : ActionPort  ActionPortLabel=if(u1 > -0.05 & u2 > 0)
  Clock : Clock
  Compare To Constant : simulink/Logic and Bit Operations/Compare To Constant  relop=<=  const=5  OutDataTypeStr=boolean
  Product : Product
  Out1 : Outport
  wires:
  Thrust/1 -> Product/1
  Product/1 -> Out1/1
  Clock/1 -> Compare To Constant/1
  Compare To Constant/1 -> Product/2

== system hopper_6dof_NED_v2_simplified/Wind Forces/Disabled ==
  Ve : Inport
  cg : Inport  Port=2
  Term1 : Terminator
  Term2 : Terminator
  Zero1 : Constant  Value=[0 0 0]
  Zero2 : Constant  Value=[0 0 0]
  Fxyz_wind : Outport
  Mxyz_wind : Outport  Port=2
  wires:
  Ve/1 -> Term1/1
  cg/1 -> Term2/1
  Zero1/1 -> Fxyz_wind/1
  Zero2/1 -> Mxyz_wind/1

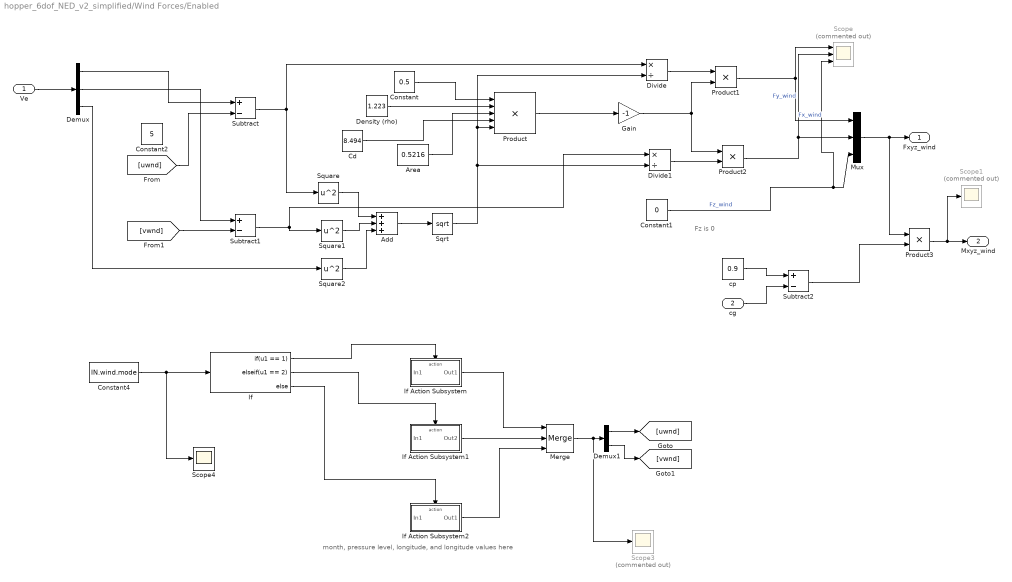
== system hopper_6dof_NED_v2_simplified/Wind Forces/Enabled ==
  note: Fz is 0
  note: month, pressure level, longitude, and longitude values here
  Ve : Inport
  cg : Inport  Port=2
  Add : Sum  Inputs=+++
  Area : Constant  Value=0.5216
  Cd : Constant  Value=8.494
  Constant : Constant  Value=0.5
  Constant1 : Constant  Value=0
  Constant2 : Constant  Value=5
  Constant4 : Constant  Value=IN.wind.mode
  Demux : Demux  Outputs=3
  Demux1 : Demux  Outputs=2
  Density (rho) : Constant  Value=1.223
  Divide : Product  Inputs=*/
  Divide1 : Product  Inputs=*/
  Gain : Gain  Gain=-1
  If : If  IfExpression=u1 == 1  ElseIfExpressions=u1 == 2
  If Action Subsystem : Subsystem  TreatAsAtomicUnit=on
  If Action Subsystem1 : Subsystem  TreatAsAtomicUnit=on
  If Action Subsystem2 : Subsystem  TreatAsAtomicUnit=on
  Merge : Merge  Inputs=3
  Mux : Mux  Inputs=3
  Product : Product  Inputs=5
  Product1 : Product
  Product2 : Product
  Product3 : Product
  Scope : Scope  Commented=on  NumInputPorts=3
      settings: ActiveDisplayYMinimum=-3.3865408119999993  ActiveDisplayYMaximum=30.478867308  DataLoggingVariableName=ScopeData58
  Scope1 : Scope  Commented=on
      settings: ActiveDisplayYMinimum=-10.256382918668168  ActiveDisplayYMaximum=17.46231209617951  DataLoggingVariableName=ScopeData89
  Scope3 : Scope  Commented=on
      settings: ActiveDisplayYMinimum=4  ActiveDisplayYMaximum=6  DataLoggingVariableName=ScopeData90
  Scope4 : Scope
      settings: ActiveDisplayYMinimum=1  ActiveDisplayYMaximum=3  DataLoggingVariableName=ScopeData91
  Sqrt : Sqrt
  Square : Math  Operator=square
  Square1 : Math  Operator=square
  Square2 : Math  Operator=square
  Subtract : Sum  Inputs=+-
  Subtract1 : Sum  Inputs=+-
  Subtract2 : Sum  Inputs=+-
  cp : Constant  Value=0.9
  Fxyz_wind : Outport
  Mxyz_wind : Outport  Port=2
  wires:
  Demux/1 -> Subtract/1
  Square1/1 -> Add/2
  Product/1 -> Gain/1
  Add/1 -> Sqrt/1
  Divide/1 -> Product1/1
  If Action Subsystem1/1(Out2) -> Merge/2
  Demux/2 -> Subtract1/1
  Constant/1 -> Product/1
  If Action Subsystem2/1(Out1) -> Merge/3
  cg/1 -> Subtract2/2
  If Action Subsystem/1(Out1) -> Merge/1
  Density (rho)/1 -> Product/2
  Subtract1/1 -> Divide1/1, Square1/1
  Cd/1 -> Product/4
  Product1/1 -> Mux/1, Scope/1  "Fx_wind"
  If/3 -> If Action Subsystem2/Action
  Constant1/1 -> Mux/3, Scope/3  "Fz_wind"
  Constant4/1 -> If/1, Scope4/1
  Product2/1 -> Mux/2, Scope/2  "Fy_wind"
  Square2/1 -> Add/3
  Area/1 -> Product/3
  [uwnd] -> Subtract/2
  Demux1/1 -> [uwnd]
  Sqrt/1 -> Product/5, Divide/2, Divide1/2
  If/2 -> If Action Subsystem1/Action
  Subtract/1 -> Square/1, Divide/1
  Ve/1 -> Demux/1
  Subtract2/1 -> Product3/2
  Gain/1 -> Product2/1, Product1/2
  Product3/1 -> Mxyz_wind/1, Scope1/1
  Demux1/2 -> [vwnd]
  Merge/1 -> Demux1/1, Scope3/1
  Square/1 -> Add/1
  Divide1/1 -> Product2/2
  cp/1 -> Subtract2/1
  Demux/3 -> Square2/1
  [vwnd] -> Subtract1/2
  Mux/1 -> Fxyz_wind/1, Product3/1
  If/1 -> If Action Subsystem/Action

== system hopper_6dof_NED_v2_simplified/Fluid Network2/COPV/COPV Leakage ==
  Leak Rate : fl_lib/Gas/Elements/Flow Resistance (G)  delta_p_nominal=0.001 MPa  mdot_nominal=0.0000000001 kg/s  rho_nominal=0 kg/m^3  area=0.01 m^2  laminar_fraction=1e-3
  Mass & Energy Flow Rate Sensor (G)2 : fl_lib/Gas/Sensors/Flow Rate Sensor (G)  mass_flow_measure=true  volumetric_flow_measure=false  volumetric_flow_conditions=foundation.enum.volumetric_flow_conditions.actual  p_std=0.101325 MPa  T_std=20 degC  energy_flow_measure=true
  PS-Simulink Converter7 : nesl_utility/PS-Simulink Converter  PhysicalDomain=network_engine_domain  SubClassName=ps_output  LeftPortType=input  RightPortType=output  PseudoPeriodic=off  Frequencies=[]  VectorFormat=inherit  Unit=inherit  AffineConversion=off
  Pressurant Mass Leak Rate : Scope  Commented=on
      settings: ActiveDisplayYMinimum=-1  ActiveDisplayYMaximum=1
  Reservoir (G) : fl_lib/Gas/Elements/Reservoir (G)  pressure_input=false  pressure_spec=foundation.enum.pressure_spec.atmospheric  reservoir_pressure=0.101325 MPa  temperature_input=false  reservoir_temperature=293.15 K  area_A=0.01 m^2  input_error_spec=foundation.enum.input_range_error.warn
  Conn1 : PMIOPort  Side=Right
  wires:
  PS-Simulink Converter7/1 -> Pressurant Mass Leak Rate/1
  connections:
  Conn1/RConn1 -- Leak Rate/RConn1
  Leak Rate/LConn1 -- Mass & Energy Flow Rate Sensor (G)2/LConn1
  Mass & Energy Flow Rate Sensor (G)2/RConn1 -- Reservoir (G)/LConn1
  Mass & Energy Flow Rate Sensor (G)2/RConn2 -- PS-Simulink Converter7/LConn1

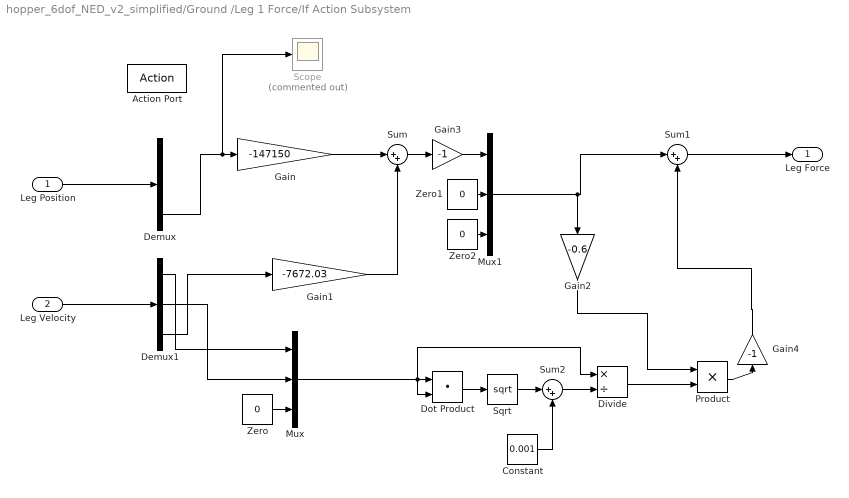
== system hopper_6dof_NED_v2_simplified/Ground /Leg 1 Force/If Action Subsystem ==
  Leg Position : Inport
  Leg Velocity : Inport  Port=2
  Action Port : ActionPort  ActionPortLabel=|
      | if(u1 > -0.001 
      | )
  Constant : Constant  Value=0.001
  Demux : Demux  Outputs=3
  Demux1 : Demux  Outputs=3
  Divide : Product  Inputs=*/
  Dot Product : DotProduct  OutDataTypeStr=Inherit: Inherit via internal rule
  Gain : Gain  Gain=-147150
  Gain1 : Gain  Gain=-7672.03
  Gain2 : Gain  Gain=-0.6
  Gain3 : Gain  Gain=-1
  Gain4 : Gain  Gain=-1
  Mux : Mux  Inputs=3
  Mux1 : Mux  Inputs=3
  Product : Product
  Scope : Scope  Commented=on
      settings: ActiveDisplayYMinimum=-1  ActiveDisplayYMaximum=1  DataLoggingVariableName=ScopeData69
  Sqrt : Sqrt
  Sum : Sum  Inputs=|++
  Sum1 : Sum  Inputs=|++
  Sum2 : Sum  Inputs=|++
  Zero : Constant  Value=0  OutDataTypeStr=Inherit: Inherit via back propagation
  Zero1 : Constant  Value=0  OutDataTypeStr=Inherit: Inherit via back propagation
  Zero2 : Constant  Value=0  OutDataTypeStr=Inherit: Inherit via back propagation
  Leg Force : Outport
  wires:
  Leg Position/1 -> Demux/1
  Leg Velocity/1 -> Demux1/1
  Gain/1 -> Sum/1
  Gain1/1 -> Sum/2
  Demux1/3 -> Gain1/1
  Demux1/2 -> Mux/2
  Demux1/1 -> Mux/1
  Mux/1 -> Dot Product/2, Dot Product/1, Divide/1
  Dot Product/1 -> Sqrt/1
  Divide/1 -> Product/2
  Gain2/1 -> Product/1
  Product/1 -> Gain4/1
  Sum1/1 -> Leg Force/1
  Sqrt/1 -> Sum2/1
  Sum2/1 -> Divide/2
  Constant/1 -> Sum2/2
  Sum/1 -> Gain3/1
  Zero1/1 -> Mux1/2
  Zero2/1 -> Mux1/3
  Mux1/1 -> Sum1/1, Gain2/1
  Demux/3 -> Scope/1, Gain/1
  Zero/1 -> Mux/3
  Gain3/1 -> Mux1/1
  Gain4/1 -> Sum1/2

== system hopper_6dof_NED_v2_simplified/Ground /Leg 1 Force/If Action Subsystem1 ==
  Action Port : ActionPort  ActionPortLabel=else
  Constant : Constant  Value=[0 0 0]
  Out1 : Outport
  wires:
  Constant/1 -> Out1/1

== system hopper_6dof_NED_v2_simplified/Ground /Leg 1 Force1/If Action Subsystem ==
  Leg Position : Inport
  Leg Velocity : Inport  Port=2
  Action Port : ActionPort  ActionPortLabel=|
      | if(u1 > -0.001 
      | )
  Constant : Constant  Value=0.001
  Demux : Demux  Outputs=3
  Demux1 : Demux  Outputs=3
  Divide : Product  Inputs=*/
  Dot Product : DotProduct  OutDataTypeStr=Inherit: Inherit via internal rule
  Gain : Gain  Gain=-147150
  Gain1 : Gain  Gain=-7672.03
  Gain2 : Gain  Gain=-0.6
  Gain3 : Gain  Gain=-1
  Gain4 : Gain  Gain=-1
  Mux : Mux  Inputs=3
  Mux1 : Mux  Inputs=3
  Product : Product
  Sqrt : Sqrt
  Sum : Sum  Inputs=|++
  Sum1 : Sum  Inputs=|++
  Sum2 : Sum  Inputs=|++
  Zero : Constant  Value=0  OutDataTypeStr=Inherit: Inherit via back propagation
  Zero1 : Constant  Value=0  OutDataTypeStr=Inherit: Inherit via back propagation
  Zero2 : Constant  Value=0  OutDataTypeStr=Inherit: Inherit via back propagation
  Leg Force : Outport
  wires:
  Leg Position/1 -> Demux/1
  Leg Velocity/1 -> Demux1/1
  Gain/1 -> Sum/1
  Gain1/1 -> Sum/2
  Demux1/3 -> Gain1/1
  Demux1/2 -> Mux/2
  Demux1/1 -> Mux/1
  Mux/1 -> Dot Product/2, Dot Product/1, Divide/1
  Dot Product/1 -> Sqrt/1
  Divide/1 -> Product/2
  Gain2/1 -> Product/1
  Product/1 -> Gain4/1
  Sum1/1 -> Leg Force/1
  Sqrt/1 -> Sum2/1
  Sum2/1 -> Divide/2
  Constant/1 -> Sum2/2
  Sum/1 -> Gain3/1
  Zero1/1 -> Mux1/2
  Zero2/1 -> Mux1/3
  Mux1/1 -> Sum1/1, Gain2/1
  Demux/3 -> Gain/1
  Zero/1 -> Mux/3
  Gain3/1 -> Mux1/1
  Gain4/1 -> Sum1/2

== system hopper_6dof_NED_v2_simplified/Ground /Leg 1 Force1/If Action Subsystem1 ==
  Action Port : ActionPort  ActionPortLabel=else
  Constant : Constant  Value=[0 0 0]
  Out1 : Outport
  wires:
  Constant/1 -> Out1/1

== system hopper_6dof_NED_v2_simplified/Ground /Leg 1 Force2/If Action Subsystem ==
  Leg Position : Inport
  Leg Velocity : Inport  Port=2
  Action Port : ActionPort  ActionPortLabel=|
      | if(u1 > -0.001 
      | )
  Constant : Constant  Value=0.001
  Demux : Demux  Outputs=3
  Demux1 : Demux  Outputs=3
  Divide : Product  Inputs=*/
  Dot Product : DotProduct  OutDataTypeStr=Inherit: Inherit via internal rule
  Gain : Gain  Gain=-147150
  Gain1 : Gain  Gain=-7672.03
  Gain2 : Gain  Gain=-0.6
  Gain3 : Gain  Gain=-1
  Gain4 : Gain  Gain=-1
  Mux : Mux  Inputs=3
  Mux1 : Mux  Inputs=3
  Product : Product
  Sqrt : Sqrt
  Sum : Sum  Inputs=|++
  Sum1 : Sum  Inputs=|++
  Sum2 : Sum  Inputs=|++
  Zero : Constant  Value=0  OutDataTypeStr=Inherit: Inherit via back propagation
  Zero1 : Constant  Value=0  OutDataTypeStr=Inherit: Inherit via back propagation
  Zero2 : Constant  Value=0  OutDataTypeStr=Inherit: Inherit via back propagation
  Leg Force : Outport
  wires:
  Leg Position/1 -> Demux/1
  Leg Velocity/1 -> Demux1/1
  Gain/1 -> Sum/1
  Gain1/1 -> Sum/2
  Demux1/3 -> Gain1/1
  Demux1/2 -> Mux/2
  Demux1/1 -> Mux/1
  Mux/1 -> Dot Product/2, Dot Product/1, Divide/1
  Dot Product/1 -> Sqrt/1
  Divide/1 -> Product/2
  Gain2/1 -> Product/1
  Product/1 -> Gain4/1
  Sum1/1 -> Leg Force/1
  Sqrt/1 -> Sum2/1
  Sum2/1 -> Divide/2
  Constant/1 -> Sum2/2
  Sum/1 -> Gain3/1
  Zero1/1 -> Mux1/2
  Zero2/1 -> Mux1/3
  Mux1/1 -> Sum1/1, Gain2/1
  Demux/3 -> Gain/1
  Zero/1 -> Mux/3
  Gain3/1 -> Mux1/1
  Gain4/1 -> Sum1/2

== system hopper_6dof_NED_v2_simplified/Ground /Leg 1 Force2/If Action Subsystem1 ==
  Action Port : ActionPort  ActionPortLabel=else
  Constant : Constant  Value=[0 0 0]
  Out1 : Outport
  wires:
  Constant/1 -> Out1/1
